simulink model "HPP"  (R2026a)
settings: Solver=ode1  StopTime=p.sim.Tstop  FixedStep=HPP_Tnet
model workspace (MAT data in the model file):
  HPP_Tnet = 0.001
  HPP_Ts = 0.001
  HPP_delays = 1
  HPP_f0 = 50
  HPP_network = 1
  HPP_simscape = 1
  buildInfo : object (value not decoded)
undefined symbols (not defined in the file): p
libraries: ee_lib x57, nesl_utility x29, fl_lib x6
(part 2 of 5)

== system HPP/HPP controller/P_set_bess to W link ==
  In1 : Inport
  gain 1 : Gain  Gain=p.ctrl.hppc.Pbase
  Out1 : Outport
  wires:
  In1/1 -> gain 1/1
  gain 1/1 -> Out1/1

== system HPP/HPP controller/P_set_spp to W link ==
  In1 : Inport
  gain 1 : Gain  Gain=p.ctrl.hppc.Pbase
  Out1 : Outport
  wires:
  In1/1 -> gain 1/1
  gain 1/1 -> Out1/1

== system HPP/HPP controller/P_set_wpp to W link ==
  In1 : Inport
  gain 1 : Gain  Gain=p.ctrl.hppc.Pbase
  Out1 : Outport
  wires:
  In1/1 -> gain 1/1
  gain 1/1 -> Out1/1

== system HPP/HPP controller/P_spp link ==
  In1 : Inport
  delay 3 : Subsystem  Description=Communication delay of p.comm.steps.meas_hppc steps, chosen per run: Fixed (HPP_delays = 1, length fixed at compile time, fastest) or Variable (HPP_delays = 2, tunable up to p.comm.maxDelay). See commParameters, comm.delays.  Variant=on
  gain 1 : Gain  Gain=1/p.ctrl.hppc.Pbase
  memory 2 : Memory
  Out1 : Outport
  wires:
  In1/1 -> gain 1/1
  memory 2/1 -> delay 3/1(u)
  gain 1/1 -> memory 2/1
  delay 3/1(y) -> Out1/1

== system HPP/HPP controller/P_wpp link ==
  In1 : Inport
  delay 3 : Subsystem  Description=Communication delay of p.comm.steps.meas_hppc steps, chosen per run: Fixed (HPP_delays = 1, length fixed at compile time, fastest) or Variable (HPP_delays = 2, tunable up to p.comm.maxDelay). See commParameters, comm.delays.  Variant=on
  gain 1 : Gain  Gain=1/p.ctrl.hppc.Pbase
  memory 2 : Memory
  Out1 : Outport
  wires:
  In1/1 -> gain 1/1
  delay 3/1(y) -> Out1/1
  memory 2/1 -> delay 3/1(u)
  gain 1/1 -> memory 2/1

== system HPP/HPP controller/Q_bess link ==
  In1 : Inport
  delay 3 : Subsystem  Description=Communication delay of p.comm.steps.meas_hppc steps, chosen per run: Fixed (HPP_delays = 1, length fixed at compile time, fastest) or Variable (HPP_delays = 2, tunable up to p.comm.maxDelay). See commParameters, comm.delays.  Variant=on
  gain 1 : Gain  Gain=1/p.ctrl.hppc.Pbase
  memory 2 : Memory
  Out1 : Outport
  wires:
  In1/1 -> gain 1/1
  gain 1/1 -> memory 2/1
  delay 3/1(y) -> Out1/1
  memory 2/1 -> delay 3/1(u)

== system HPP/HPP controller/Q_poc link ==
  In1 : Inport
  delay 3 : Subsystem  Description=Communication delay of p.comm.steps.meas_hppc steps, chosen per run: Fixed (HPP_delays = 1, length fixed at compile time, fastest) or Variable (HPP_delays = 2, tunable up to p.comm.maxDelay). See commParameters, comm.delays.  Variant=on
  gain 1 : Gain  Gain=1/p.ctrl.hppc.Pbase
  memory 2 : Memory
  Out1 : Outport
  wires:
  In1/1 -> gain 1/1
  delay 3/1(y) -> Out1/1
  memory 2/1 -> delay 3/1(u)
  gain 1/1 -> memory 2/1

== system HPP/HPP controller/Q_ref link ==
  In1 : Inport
  delay 2 : Subsystem  Description=Communication delay of p.comm.steps.tso steps, chosen per run: Fixed (HPP_delays = 1, length fixed at compile time, fastest) or Variable (HPP_delays = 2, tunable up to p.comm.maxDelay). See commParameters, comm.delays.  Variant=on
  gain 1 : Gain  Gain=1/p.ctrl.hppc.Pbase
  Out1 : Outport
  wires:
  In1/1 -> gain 1/1
  gain 1/1 -> delay 2/1(u)
  delay 2/1(y) -> Out1/1

== system HPP/HPP controller/Q_sat_bess link ==
  In1 : Inport
  delay 2 : Subsystem  Description=Communication delay of p.comm.steps.meas_hppc steps, chosen per run: Fixed (HPP_delays = 1, length fixed at compile time, fastest) or Variable (HPP_delays = 2, tunable up to p.comm.maxDelay). See commParameters, comm.delays.  Variant=on
  memory 1 : Memory
  Out1 : Outport
  wires:
  In1/1 -> memory 1/1
  delay 2/1(y) -> Out1/1
  memory 1/1 -> delay 2/1(u)

== system HPP/HPP controller/Q_sat_spp link ==
  In1 : Inport
  delay 2 : Subsystem  Description=Communication delay of p.comm.steps.meas_hppc steps, chosen per run: Fixed (HPP_delays = 1, length fixed at compile time, fastest) or Variable (HPP_delays = 2, tunable up to p.comm.maxDelay). See commParameters, comm.delays.  Variant=on
  memory 1 : Memory
  Out1 : Outport
  wires:
  In1/1 -> memory 1/1
  delay 2/1(y) -> Out1/1
  memory 1/1 -> delay 2/1(u)

== system HPP/HPP controller/Q_sat_wpp link ==
  In1 : Inport
  delay 2 : Subsystem  Description=Communication delay of p.comm.steps.meas_hppc steps, chosen per run: Fixed (HPP_delays = 1, length fixed at compile time, fastest) or Variable (HPP_delays = 2, tunable up to p.comm.maxDelay). See commParameters, comm.delays.  Variant=on
  memory 1 : Memory
  Out1 : Outport
  wires:
  In1/1 -> memory 1/1
  delay 2/1(y) -> Out1/1
  memory 1/1 -> delay 2/1(u)

== system HPP/HPP controller/Q_set_bess to var link ==
  In1 : Inport
  gain 1 : Gain  Gain=p.ctrl.hppc.Pbase
  Out1 : Outport
  wires:
  In1/1 -> gain 1/1
  gain 1/1 -> Out1/1

== system HPP/HPP controller/Q_set_spp to var link ==
  In1 : Inport
  gain 1 : Gain  Gain=p.ctrl.hppc.Pbase
  Out1 : Outport
  wires:
  In1/1 -> gain 1/1
  gain 1/1 -> Out1/1

== system HPP/HPP controller/Q_set_wpp to var link ==
  In1 : Inport
  gain 1 : Gain  Gain=p.ctrl.hppc.Pbase
  Out1 : Outport
  wires:
  In1/1 -> gain 1/1
  gain 1/1 -> Out1/1

== system HPP/HPP controller/Q_spp link ==
  In1 : Inport
  delay 3 : Subsystem  Description=Communication delay of p.comm.steps.meas_hppc steps, chosen per run: Fixed (HPP_delays = 1, length fixed at compile time, fastest) or Variable (HPP_delays = 2, tunable up to p.comm.maxDelay). See commParameters, comm.delays.  Variant=on
  gain 1 : Gain  Gain=1/p.ctrl.hppc.Pbase
  memory 2 : Memory
  Out1 : Outport
  wires:
  In1/1 -> gain 1/1
  delay 3/1(y) -> Out1/1
  memory 2/1 -> delay 3/1(u)
  gain 1/1 -> memory 2/1

== system HPP/HPP controller/Q_wpp link ==
  In1 : Inport
  delay 3 : Subsystem  Description=Communication delay of p.comm.steps.meas_hppc steps, chosen per run: Fixed (HPP_delays = 1, length fixed at compile time, fastest) or Variable (HPP_delays = 2, tunable up to p.comm.maxDelay). See commParameters, comm.delays.  Variant=on
  gain 1 : Gain  Gain=1/p.ctrl.hppc.Pbase
  memory 2 : Memory
  Out1 : Outport
  wires:
  In1/1 -> gain 1/1
  memory 2/1 -> delay 3/1(u)
  gain 1/1 -> memory 2/1
  delay 3/1(y) -> Out1/1

== system HPP/HPP controller/SOC_bess link ==
  In1 : Inport
  delay 2 : Subsystem  Description=Communication delay of p.comm.steps.meas_hppc steps, chosen per run: Fixed (HPP_delays = 1, length fixed at compile time, fastest) or Variable (HPP_delays = 2, tunable up to p.comm.maxDelay). See commParameters, comm.delays.  Variant=on
  memory 1 : Memory
  Out1 : Outport
  wires:
  In1/1 -> memory 1/1
  delay 2/1(y) -> Out1/1
  memory 1/1 -> delay 2/1(u)

== system HPP/HPP controller/V_poc link ==
  In1 : Inport
  delay 2 : Subsystem  Description=Communication delay of p.comm.steps.meas_hppc steps, chosen per run: Fixed (HPP_delays = 1, length fixed at compile time, fastest) or Variable (HPP_delays = 2, tunable up to p.comm.maxDelay). See commParameters, comm.delays.  Variant=on
  memory 1 : Memory
  Out1 : Outport
  wires:
  In1/1 -> memory 1/1
  memory 1/1 -> delay 2/1(u)
  delay 2/1(y) -> Out1/1

== system HPP/Network/Grid frequency ==
  POC meas : Inport
  1 + w : Bias  Bias=1  SaturateOnIntegerOverflow=off
  HPP change : Subsystem  Description=dPh = (P_poc - P_hold) / Ssys; P_hold follows P_poc until tOn (system balanced at tOn)
  POC sel : BusSelector  OutputSignals=P_poc
  P_poc[k-1] : UnitDelay  SampleTime=-1
  active : Subsystem  Description=swing equation on (swing = 1) and t >= tOn
  disturbance : Subsystem  Description=dP_dist = dist.dP for t >= dist.t0
  grid source angle : Subsystem  Description=th = wrap(th[k-1] + 2 pi f0 (f - 1) Ts); theta = wrap(th + dphi (t >= pjump.t0))
  imposed : Subsystem  Description=1 + fev.df (t >= fev.t0) + profile(t)
  swing : Constant  Value=g.sys.swing
  swing equation : Subsystem  Description=2H dw/dt = Pm + dPh - dP_dist - D w; governor and turbine (Pm); forward Euler from tOn
  swing? : Switch  Criteria=u2 > Threshold  Threshold=0.5  SaturateOnIntegerOverflow=off  InputSameDT=off
  t : DigitalClock  SampleTime=p.sim.Ts
  f : Outport
  theta : Outport  Port=2
  wires:
  POC meas/1 -> POC sel/1
  POC sel/1 -> P_poc[k-1]/1  "<P_poc>"
  P_poc[k-1]/1 -> HPP change/1(P_poc)  "P_poc"
  t/1 -> active/1(t), disturbance/1(t), imposed/1(t), grid source angle/2(t)  "t"
  active/1(active) -> HPP change/2(active), swing equation/3(active)  "active"
  HPP change/1(dPh) -> swing equation/1(dPh)  "dPh"
  disturbance/1(dPd) -> swing equation/2(dPd)  "dPd"
  swing equation/1(w) -> 1 + w/1  "w"
  1 + w/1 -> swing?/1
  swing/1 -> swing?/2
  imposed/1(f_imp) -> swing?/3  "f_imp"
  swing?/1 -> f/1, grid source angle/1(f)  "f"
  grid source angle/1(theta) -> theta/1  "theta"

== system HPP/Network/Network model ==
  note: 1) Add Subsystem or Model blocks as valid variant choices.
      | 2) You cannot connect blocks at this level. At simulation, connectivity is automatically
      | determined, based on the active variant and port name matching.
  I wpp : Inport
  I spp : Inport  Port=2
  I bess : Inport  Port=3
  f grid : Inport  Port=4
  theta : Inport  Port=5
  Nodal : Subsystem  VariantControl=HPP_network == 1  mask{net=p.net.solver}
      mask prompts: net "Network solver data"
      mask help: Positive-sequence phasor network (collector system, transformers, grid). Solves V = Z*I each step. Data from networkSolverData(p).
  Simscape : Subsystem  Description=Network as a Simscape Electrical model in phasor (frequency-and-time) or EMT mode (buildNetworkSimscape). Same ports as the nodal network. Electrical nodes are joined by Connection Labels (collector, tap, HPP bus, POC); signals by local Goto/From.  VariantControl=HPP_network == 2
  network : Outport
  POC meas : Outport  Port=2

== system HPP/PV plant/I_im to system pu link ==
  In1 : Inport
  gain 1 : Gain  Gain=p.ctrl.pv.Pbase/p.grid.Pbase
  Out1 : Outport
  wires:
  gain 1/1 -> Out1/1
  In1/1 -> gain 1/1

== system HPP/PV plant/I_re to system pu link ==
  In1 : Inport
  gain 1 : Gain  Gain=p.ctrl.pv.Pbase/p.grid.Pbase
  Out1 : Outport
  wires:
  In1/1 -> gain 1/1
  gain 1/1 -> Out1/1

== system HPP/PV plant/P to W link ==
  In1 : Inport
  gain 1 : Gain  Gain=p.ctrl.sppc.Pbase
  Out1 : Outport
  wires:
  gain 1/1 -> Out1/1
  In1/1 -> gain 1/1

== system HPP/PV plant/P_avail to W link ==
  In1 : Inport
  gain 1 : Gain  Gain=p.ctrl.sppc.Pbase
  Out1 : Outport
  wires:
  gain 1/1 -> Out1/1
  In1/1 -> gain 1/1

== system HPP/PV plant/P_avail_k link ==
  In1 : Inport
  delay 3 : Subsystem  Description=Communication delay of p.comm.steps.meas_plant steps, chosen per run: Fixed (HPP_delays = 1, length fixed at compile time, fastest) or Variable (HPP_delays = 2, tunable up to p.comm.maxDelay). See commParameters, comm.delays.  Variant=on
  gain 1 : Gain  Gain=p.ctrl.pv.Pbase/p.ctrl.sppc.Pbase
  memory 2 : Memory
  Out1 : Outport
  wires:
  In1/1 -> gain 1/1
  gain 1/1 -> memory 2/1
  memory 2/1 -> delay 3/1(u)
  delay 3/1(y) -> Out1/1

== system HPP/PV plant/P_meas link ==
  In1 : Inport
  delay 3 : Subsystem  Description=Communication delay of p.comm.steps.meas_plant steps, chosen per run: Fixed (HPP_delays = 1, length fixed at compile time, fastest) or Variable (HPP_delays = 2, tunable up to p.comm.maxDelay). See commParameters, comm.delays.  Variant=on
  gain 1 : Gain  Gain=1/p.ctrl.sppc.Pbase
  memory 2 : Memory
  Out1 : Outport
  wires:
  In1/1 -> gain 1/1
  gain 1/1 -> memory 2/1
  memory 2/1 -> delay 3/1(u)
  delay 3/1(y) -> Out1/1

== system HPP/PV plant/P_set link ==
  In1 : Inport
  delay 1 : Subsystem  Description=Communication delay of p.comm.steps.hppc_to_plant steps, chosen per run: Fixed (HPP_delays = 1, length fixed at compile time, fastest) or Variable (HPP_delays = 2, tunable up to p.comm.maxDelay). See commParameters, comm.delays.  Variant=on
  gain 2 : Gain  Gain=1/p.ctrl.sppc.Pbase
  Out1 : Outport
  wires:
  In1/1 -> delay 1/1(u)
  delay 1/1(y) -> gain 2/1
  gain 2/1 -> Out1/1

== system HPP/PV plant/P_set_k link ==
  In1 : Inport
  delay 1 : Subsystem  Description=Communication delay of p.comm.steps.plant_to_asset steps, chosen per run: Fixed (HPP_delays = 1, length fixed at compile time, fastest) or Variable (HPP_delays = 2, tunable up to p.comm.maxDelay). See commParameters, comm.delays.  Variant=on
  gain 2 : Gain  Gain=p.ctrl.sppc.Pbase/p.ctrl.pv.Pbase
  Out1 : Outport
  wires:
  In1/1 -> delay 1/1(u)
  delay 1/1(y) -> gain 2/1
  gain 2/1 -> Out1/1

== system HPP/PV plant/Q to W link ==
  In1 : Inport
  gain 1 : Gain  Gain=p.ctrl.sppc.Pbase
  Out1 : Outport
  wires:
  gain 1/1 -> Out1/1
  In1/1 -> gain 1/1

== system HPP/PV plant/Q_meas link ==
  In1 : Inport
  delay 3 : Subsystem  Description=Communication delay of p.comm.steps.meas_plant steps, chosen per run: Fixed (HPP_delays = 1, length fixed at compile time, fastest) or Variable (HPP_delays = 2, tunable up to p.comm.maxDelay). See commParameters, comm.delays.  Variant=on
  gain 1 : Gain  Gain=1/p.ctrl.sppc.Pbase
  memory 2 : Memory
  Out1 : Outport
  wires:
  In1/1 -> gain 1/1
  gain 1/1 -> memory 2/1
  memory 2/1 -> delay 3/1(u)
  delay 3/1(y) -> Out1/1

== system HPP/PV plant/Q_set link ==
  In1 : Inport
  delay 1 : Subsystem  Description=Communication delay of p.comm.steps.hppc_to_plant steps, chosen per run: Fixed (HPP_delays = 1, length fixed at compile time, fastest) or Variable (HPP_delays = 2, tunable up to p.comm.maxDelay). See commParameters, comm.delays.  Variant=on
  gain 2 : Gain  Gain=1/p.ctrl.sppc.Pbase
  Out1 : Outport
  wires:
  delay 1/1(y) -> gain 2/1
  In1/1 -> delay 1/1(u)
  gain 2/1 -> Out1/1

== system HPP/PV plant/Q_set_k link ==
  In1 : Inport
  delay 1 : Subsystem  Description=Communication delay of p.comm.steps.plant_to_asset steps, chosen per run: Fixed (HPP_delays = 1, length fixed at compile time, fastest) or Variable (HPP_delays = 2, tunable up to p.comm.maxDelay). See commParameters, comm.delays.  Variant=on
  gain 2 : Gain  Gain=p.ctrl.sppc.Pbase/p.ctrl.pv.Pbase
  Out1 : Outport
  wires:
  In1/1 -> delay 1/1(u)
  delay 1/1(y) -> gain 2/1
  gain 2/1 -> Out1/1

== system HPP/PV plant/V_meas link ==
  In1 : Inport
  delay 2 : Subsystem  Description=Communication delay of p.comm.steps.meas_plant steps, chosen per run: Fixed (HPP_delays = 1, length fixed at compile time, fastest) or Variable (HPP_delays = 2, tunable up to p.comm.maxDelay). See commParameters, comm.delays.  Variant=on
  memory 1 : Memory
  Out1 : Outport
  wires:
  In1/1 -> memory 1/1
  delay 2/1(y) -> Out1/1
  memory 1/1 -> delay 2/1(u)

== system HPP/PV plant/f_meas link ==
  In1 : Inport
  memory 1 : Memory
  Out1 : Outport
  wires:
  memory 1/1 -> Out1/1
  In1/1 -> memory 1/1

== system HPP/Wind plant/I_im to system pu link ==
  In1 : Inport
  gain 1 : Gain  Gain=p.ctrl.wt.Pbase/p.grid.Pbase
  Out1 : Outport
  wires:
  In1/1 -> gain 1/1
  gain 1/1 -> Out1/1

== system HPP/Wind plant/I_re to system pu link ==
  In1 : Inport
  gain 1 : Gain  Gain=p.ctrl.wt.Pbase/p.grid.Pbase
  Out1 : Outport
  wires:
  In1/1 -> gain 1/1
  gain 1/1 -> Out1/1

== system HPP/Wind plant/P to W link ==
  In1 : Inport
  gain 1 : Gain  Gain=p.ctrl.wppc.Pbase
  Out1 : Outport
  wires:
  gain 1/1 -> Out1/1
  In1/1 -> gain 1/1

== system HPP/Wind plant/P_avail to W link ==
  In1 : Inport
  gain 1 : Gain  Gain=p.ctrl.wppc.Pbase
  Out1 : Outport
  wires:
  gain 1/1 -> Out1/1
  In1/1 -> gain 1/1

== system HPP/Wind plant/P_avail_k link ==
  In1 : Inport
  delay 3 : Subsystem  Description=Communication delay of p.comm.steps.meas_plant steps, chosen per run: Fixed (HPP_delays = 1, length fixed at compile time, fastest) or Variable (HPP_delays = 2, tunable up to p.comm.maxDelay). See commParameters, comm.delays.  Variant=on
  gain 1 : Gain  Gain=p.ctrl.wt.Pbase/p.ctrl.wppc.Pbase
  memory 2 : Memory
  Out1 : Outport
  wires:
  In1/1 -> gain 1/1
  gain 1/1 -> memory 2/1
  memory 2/1 -> delay 3/1(u)
  delay 3/1(y) -> Out1/1

== system HPP/Wind plant/P_meas link ==
  In1 : Inport
  delay 3 : Subsystem  Description=Communication delay of p.comm.steps.meas_plant steps, chosen per run: Fixed (HPP_delays = 1, length fixed at compile time, fastest) or Variable (HPP_delays = 2, tunable up to p.comm.maxDelay). See commParameters, comm.delays.  Variant=on
  gain 1 : Gain  Gain=1/p.ctrl.wppc.Pbase
  memory 2 : Memory
  Out1 : Outport
  wires:
  In1/1 -> gain 1/1
  gain 1/1 -> memory 2/1
  memory 2/1 -> delay 3/1(u)
  delay 3/1(y) -> Out1/1

== system HPP/Wind plant/P_set link ==
  In1 : Inport
  delay 1 : Subsystem  Description=Communication delay of p.comm.steps.hppc_to_plant steps, chosen per run: Fixed (HPP_delays = 1, length fixed at compile time, fastest) or Variable (HPP_delays = 2, tunable up to p.comm.maxDelay). See commParameters, comm.delays.  Variant=on
  gain 2 : Gain  Gain=1/p.ctrl.wppc.Pbase
  Out1 : Outport
  wires:
  In1/1 -> delay 1/1(u)
  delay 1/1(y) -> gain 2/1
  gain 2/1 -> Out1/1

== system HPP/Wind plant/P_set_k link ==
  In1 : Inport
  delay 1 : Subsystem  Description=Communication delay of p.comm.steps.plant_to_asset steps, chosen per run: Fixed (HPP_delays = 1, length fixed at compile time, fastest) or Variable (HPP_delays = 2, tunable up to p.comm.maxDelay). See commParameters, comm.delays.  Variant=on
  gain 2 : Gain  Gain=p.ctrl.wppc.Pbase/p.ctrl.wt.Pbase
  Out1 : Outport
  wires:
  In1/1 -> delay 1/1(u)
  delay 1/1(y) -> gain 2/1
  gain 2/1 -> Out1/1

== system HPP/Wind plant/Q to W link ==
  In1 : Inport
  gain 1 : Gain  Gain=p.ctrl.wppc.Pbase
  Out1 : Outport
  wires:
  In1/1 -> gain 1/1
  gain 1/1 -> Out1/1

== system HPP/Wind plant/Q_meas link ==
  In1 : Inport
  delay 3 : Subsystem  Description=Communication delay of p.comm.steps.meas_plant steps, chosen per run: Fixed (HPP_delays = 1, length fixed at compile time, fastest) or Variable (HPP_delays = 2, tunable up to p.comm.maxDelay). See commParameters, comm.delays.  Variant=on
  gain 1 : Gain  Gain=1/p.ctrl.wppc.Pbase
  memory 2 : Memory
  Out1 : Outport
  wires:
  In1/1 -> gain 1/1
  gain 1/1 -> memory 2/1
  memory 2/1 -> delay 3/1(u)
  delay 3/1(y) -> Out1/1

== system HPP/Wind plant/Q_set link ==
  In1 : Inport
  delay 1 : Subsystem  Description=Communication delay of p.comm.steps.hppc_to_plant steps, chosen per run: Fixed (HPP_delays = 1, length fixed at compile time, fastest) or Variable (HPP_delays = 2, tunable up to p.comm.maxDelay). See commParameters, comm.delays.  Variant=on
  gain 2 : Gain  Gain=1/p.ctrl.wppc.Pbase
  Out1 : Outport
  wires:
  In1/1 -> delay 1/1(u)
  delay 1/1(y) -> gain 2/1
  gain 2/1 -> Out1/1

== system HPP/Wind plant/Q_set_k link ==
  In1 : Inport
  delay 1 : Subsystem  Description=Communication delay of p.comm.steps.plant_to_asset steps, chosen per run: Fixed (HPP_delays = 1, length fixed at compile time, fastest) or Variable (HPP_delays = 2, tunable up to p.comm.maxDelay). See commParameters, comm.delays.  Variant=on
  gain 2 : Gain  Gain=p.ctrl.wppc.Pbase/p.ctrl.wt.Pbase
  Out1 : Outport
  wires:
  In1/1 -> delay 1/1(u)
  delay 1/1(y) -> gain 2/1
  gain 2/1 -> Out1/1

== system HPP/Wind plant/V_meas link ==
  In1 : Inport
  delay 2 : Subsystem  Description=Communication delay of p.comm.steps.meas_plant steps, chosen per run: Fixed (HPP_delays = 1, length fixed at compile time, fastest) or Variable (HPP_delays = 2, tunable up to p.comm.maxDelay). See commParameters, comm.delays.  Variant=on
  memory 1 : Memory
  Out1 : Outport
  wires:
  In1/1 -> memory 1/1
  memory 1/1 -> delay 2/1(u)
  delay 2/1(y) -> Out1/1

== system HPP/Wind plant/f_meas link ==
  In1 : Inport
  memory 1 : Memory
  Out1 : Outport
  wires:
  In1/1 -> memory 1/1
  memory 1/1 -> Out1/1

== system HPP/BESS plant/P_avail_k link/delay 3 ==
  note: 1) Add Subsystem or Model blocks as valid variant choices.
      | 2) You cannot connect blocks at this level. At simulation, connectivity is automatically
      | determined, based on the active variant and port name matching.
  u : Inport
  Fixed : Subsystem  VariantControl=HPP_delays == 1
  Variable : Subsystem  VariantControl=HPP_delays == 2
  y : Outport

== system HPP/BESS plant/P_meas link/delay 3 ==
  note: 1) Add Subsystem or Model blocks as valid variant choices.
      | 2) You cannot connect blocks at this level. At simulation, connectivity is automatically
      | determined, based on the active variant and port name matching.
  u : Inport
  Fixed : Subsystem  VariantControl=HPP_delays == 1
  Variable : Subsystem  VariantControl=HPP_delays == 2
  y : Outport

== system HPP/BESS plant/P_set link/delay 1 ==
  note: 1) Add Subsystem or Model blocks as valid variant choices.
      | 2) You cannot connect blocks at this level. At simulation, connectivity is automatically
      | determined, based on the active variant and port name matching.
  u : Inport
  Fixed : Subsystem  VariantControl=HPP_delays == 1
  Variable : Subsystem  VariantControl=HPP_delays == 2
  y : Outport

== system HPP/BESS plant/P_set_k link/delay 1 ==
  note: 1) Add Subsystem or Model blocks as valid variant choices.
      | 2) You cannot connect blocks at this level. At simulation, connectivity is automatically
      | determined, based on the active variant and port name matching.
  u : Inport
  Fixed : Subsystem  VariantControl=HPP_delays == 1
  Variable : Subsystem  VariantControl=HPP_delays == 2
  y : Outport

== system HPP/BESS plant/Q_meas link/delay 3 ==
  note: 1) Add Subsystem or Model blocks as valid variant choices.
      | 2) You cannot connect blocks at this level. At simulation, connectivity is automatically
      | determined, based on the active variant and port name matching.
  u : Inport
  Fixed : Subsystem  VariantControl=HPP_delays == 1
  Variable : Subsystem  VariantControl=HPP_delays == 2
  y : Outport

== system HPP/BESS plant/Q_set link/delay 1 ==
  note: 1) Add Subsystem or Model blocks as valid variant choices.
      | 2) You cannot connect blocks at this level. At simulation, connectivity is automatically
      | determined, based on the active variant and port name matching.
  u : Inport
  Fixed : Subsystem  VariantControl=HPP_delays == 1
  Variable : Subsystem  VariantControl=HPP_delays == 2
  y : Outport

== system HPP/BESS plant/Q_set_k link/delay 1 ==
  note: 1) Add Subsystem or Model blocks as valid variant choices.
      | 2) You cannot connect blocks at this level. At simulation, connectivity is automatically
      | determined, based on the active variant and port name matching.
  u : Inport
  Fixed : Subsystem  VariantControl=HPP_delays == 1
  Variable : Subsystem  VariantControl=HPP_delays == 2
  y : Outport

== system HPP/BESS plant/SOC_k link/delay 2 ==
  note: 1) Add Subsystem or Model blocks as valid variant choices.
      | 2) You cannot connect blocks at this level. At simulation, connectivity is automatically
      | determined, based on the active variant and port name matching.
  u : Inport
  Fixed : Subsystem  VariantControl=HPP_delays == 1
  Variable : Subsystem  VariantControl=HPP_delays == 2
  y : Outport

== system HPP/BESS plant/V_meas link/delay 2 ==
  note: 1) Add Subsystem or Model blocks as valid variant choices.
      | 2) You cannot connect blocks at this level. At simulation, connectivity is automatically
      | determined, based on the active variant and port name matching.
  u : Inport
  Fixed : Subsystem  VariantControl=HPP_delays == 1
  Variable : Subsystem  VariantControl=HPP_delays == 2
  y : Outport

== system HPP/HPP controller/P_avail_spp link/delay 3 ==
  note: 1) Add Subsystem or Model blocks as valid variant choices.
      | 2) You cannot connect blocks at this level. At simulation, connectivity is automatically
      | determined, based on the active variant and port name matching.
  u : Inport
  Fixed : Subsystem  VariantControl=HPP_delays == 1
  Variable : Subsystem  VariantControl=HPP_delays == 2
  y : Outport

== system HPP/HPP controller/P_avail_wpp link/delay 3 ==
  note: 1) Add Subsystem or Model blocks as valid variant choices.
      | 2) You cannot connect blocks at this level. At simulation, connectivity is automatically
      | determined, based on the active variant and port name matching.
  u : Inport
  Fixed : Subsystem  VariantControl=HPP_delays == 1
  Variable : Subsystem  VariantControl=HPP_delays == 2
  y : Outport

== system HPP/HPP controller/P_bess link/delay 3 ==
  note: 1) Add Subsystem or Model blocks as valid variant choices.
      | 2) You cannot connect blocks at this level. At simulation, connectivity is automatically
      | determined, based on the active variant and port name matching.
  u : Inport
  Fixed : Subsystem  VariantControl=HPP_delays == 1
  Variable : Subsystem  VariantControl=HPP_delays == 2
  y : Outport

== system HPP/HPP controller/P_chg_max_bess link/delay 3 ==
  note: 1) Add Subsystem or Model blocks as valid variant choices.
      | 2) You cannot connect blocks at this level. At simulation, connectivity is automatically
      | determined, based on the active variant and port name matching.
  u : Inport
  Fixed : Subsystem  VariantControl=HPP_delays == 1
  Variable : Subsystem  VariantControl=HPP_delays == 2
  y : Outport

== system HPP/HPP controller/P_dis_max_bess link/delay 3 ==
  note: 1) Add Subsystem or Model blocks as valid variant choices.
      | 2) You cannot connect blocks at this level. At simulation, connectivity is automatically
      | determined, based on the active variant and port name matching.
  u : Inport
  Fixed : Subsystem  VariantControl=HPP_delays == 1
  Variable : Subsystem  VariantControl=HPP_delays == 2
  y : Outport

== system HPP/HPP controller/P_poc link/delay 3 ==
  note: 1) Add Subsystem or Model blocks as valid variant choices.
      | 2) You cannot connect blocks at this level. At simulation, connectivity is automatically
      | determined, based on the active variant and port name matching.
  u : Inport
  Fixed : Subsystem  VariantControl=HPP_delays == 1
  Variable : Subsystem  VariantControl=HPP_delays == 2
  y : Outport

== system HPP/HPP controller/P_ref link/delay 2 ==
  note: 1) Add Subsystem or Model blocks as valid variant choices.
      | 2) You cannot connect blocks at this level. At simulation, connectivity is automatically
      | determined, based on the active variant and port name matching.
  u : Inport
  Fixed : Subsystem  VariantControl=HPP_delays == 1
  Variable : Subsystem  VariantControl=HPP_delays == 2
  y : Outport

== system HPP/HPP controller/P_spp link/delay 3 ==
  note: 1) Add Subsystem or Model blocks as valid variant choices.
      | 2) You cannot connect blocks at this level. At simulation, connectivity is automatically
      | determined, based on the active variant and port name matching.
  u : Inport
  Fixed : Subsystem  VariantControl=HPP_delays == 1
  Variable : Subsystem  VariantControl=HPP_delays == 2
  y : Outport

== system HPP/HPP controller/P_wpp link/delay 3 ==
  note: 1) Add Subsystem or Model blocks as valid variant choices.
      | 2) You cannot connect blocks at this level. At simulation, connectivity is automatically
      | determined, based on the active variant and port name matching.
  u : Inport
  Fixed : Subsystem  VariantControl=HPP_delays == 1
  Variable : Subsystem  VariantControl=HPP_delays == 2
  y : Outport

== system HPP/HPP controller/Q_bess link/delay 3 ==
  note: 1) Add Subsystem or Model blocks as valid variant choices.
      | 2) You cannot connect blocks at this level. At simulation, connectivity is automatically
      | determined, based on the active variant and port name matching.
  u : Inport
  Fixed : Subsystem  VariantControl=HPP_delays == 1
  Variable : Subsystem  VariantControl=HPP_delays == 2
  y : Outport

== system HPP/HPP controller/Q_poc link/delay 3 ==
  note: 1) Add Subsystem or Model blocks as valid variant choices.
      | 2) You cannot connect blocks at this level. At simulation, connectivity is automatically
      | determined, based on the active variant and port name matching.
  u : Inport
  Fixed : Subsystem  VariantControl=HPP_delays == 1
  Variable : Subsystem  VariantControl=HPP_delays == 2
  y : Outport

== system HPP/HPP controller/Q_ref link/delay 2 ==
  note: 1) Add Subsystem or Model blocks as valid variant choices.
      | 2) You cannot connect blocks at this level. At simulation, connectivity is automatically
      | determined, based on the active variant and port name matching.
  u : Inport
  Fixed : Subsystem  VariantControl=HPP_delays == 1
  Variable : Subsystem  VariantControl=HPP_delays == 2
  y : Outport

== system HPP/HPP controller/Q_sat_bess link/delay 2 ==
  note: 1) Add Subsystem or Model blocks as valid variant choices.
      | 2) You cannot connect blocks at this level. At simulation, connectivity is automatically
      | determined, based on the active variant and port name matching.
  u : Inport
  Fixed : Subsystem  VariantControl=HPP_delays == 1
  Variable : Subsystem  VariantControl=HPP_delays == 2
  y : Outport

== system HPP/HPP controller/Q_sat_spp link/delay 2 ==
  note: 1) Add Subsystem or Model blocks as valid variant choices.
      | 2) You cannot connect blocks at this level. At simulation, connectivity is automatically
      | determined, based on the active variant and port name matching.
  u : Inport
  Fixed : Subsystem  VariantControl=HPP_delays == 1
  Variable : Subsystem  VariantControl=HPP_delays == 2
  y : Outport

== system HPP/HPP controller/Q_sat_wpp link/delay 2 ==
  note: 1) Add Subsystem or Model blocks as valid variant choices.
      | 2) You cannot connect blocks at this level. At simulation, connectivity is automatically
      | determined, based on the active variant and port name matching.
  u : Inport
  Fixed : Subsystem  VariantControl=HPP_delays == 1
  Variable : Subsystem  VariantControl=HPP_delays == 2
  y : Outport

== system HPP/HPP controller/Q_spp link/delay 3 ==
  note: 1) Add Subsystem or Model blocks as valid variant choices.
      | 2) You cannot connect blocks at this level. At simulation, connectivity is automatically
      | determined, based on the active variant and port name matching.
  u : Inport
  Fixed : Subsystem  VariantControl=HPP_delays == 1
  Variable : Subsystem  VariantControl=HPP_delays == 2
  y : Outport

== system HPP/HPP controller/Q_wpp link/delay 3 ==
  note: 1) Add Subsystem or Model blocks as valid variant choices.
      | 2) You cannot connect blocks at this level. At simulation, connectivity is automatically
      | determined, based on the active variant and port name matching.
  u : Inport
  Fixed : Subsystem  VariantControl=HPP_delays == 1
  Variable : Subsystem  VariantControl=HPP_delays == 2
  y : Outport

== system HPP/HPP controller/SOC_bess link/delay 2 ==
  note: 1) Add Subsystem or Model blocks as valid variant choices.
      | 2) You cannot connect blocks at this level. At simulation, connectivity is automatically
      | determined, based on the active variant and port name matching.
  u : Inport
  Fixed : Subsystem  VariantControl=HPP_delays == 1
  Variable : Subsystem  VariantControl=HPP_delays == 2
  y : Outport

== system HPP/HPP controller/V_poc link/delay 2 ==
  note: 1) Add Subsystem or Model blocks as valid variant choices.
      | 2) You cannot connect blocks at this level. At simulation, connectivity is automatically
      | determined, based on the active variant and port name matching.
  u : Inport
  Fixed : Subsystem  VariantControl=HPP_delays == 1
  Variable : Subsystem  VariantControl=HPP_delays == 2
  y : Outport

== system HPP/Network/Grid frequency/HPP change ==
  P_poc : Inport
  active : Inport  Port=2
  P_hold[k-1] : Delay  DelayLength=1  InitialConditionSource=Input port
      settings: InputPortMap=u0,p4
  P_poc - P_hold : Sum  Inputs=+-
  Ssys : Constant  Value=g.sys.Ssys
  hold? : Switch  Criteria=u2 ~= 0  SaturateOnIntegerOverflow=off  InputSameDT=off
  ÷ Ssys : Product  Inputs=*/
  dPh : Outport
  wires:
  P_hold[k-1]/1 -> hold?/1
  active/1 -> hold?/2
  P_poc/1 -> hold?/3, P_hold[k-1]/2, P_poc - P_hold/1
  hold?/1 -> P_hold[k-1]/1, P_poc - P_hold/2  "P_hold"
  P_poc - P_hold/1 -> ÷ Ssys/1
  Ssys/1 -> ÷ Ssys/2
  ÷ Ssys/1 -> dPh/1

== system HPP/Network/Grid frequency/active ==
  t : Inport
  0.5 : Constant  Value=0.5
  and : Logic  AllPortsSameDT=off  OutDataTypeStr=boolean
  swing : Constant  Value=g.sys.swing
  swing > 0.5 : RelationalOperator  Operator=>  OutDataTypeStr=boolean  RndMeth=Simplest  InputSameDT=off
  t >= tOn : RelationalOperator  OutDataTypeStr=boolean  RndMeth=Simplest  InputSameDT=off
  tOn : Constant  Value=g.sys.tOn
  active : Outport
  wires:
  t/1 -> t >= tOn/1
  tOn/1 -> t >= tOn/2
  swing/1 -> swing > 0.5/1
  0.5/1 -> swing > 0.5/2
  t >= tOn/1 -> and/1
  swing > 0.5/1 -> and/2
  and/1 -> active/1

== system HPP/Network/Grid frequency/disturbance ==
  t : Inport
  dP : Gain  Gain=g.sys.dist.dP
  dist t0 : Constant  Value=g.sys.dist.t0
  on : DataTypeConversion  OutDataTypeStr=double  SaturateOnIntegerOverflow=off  RndMeth=Floor
  t >= t0 : RelationalOperator  OutDataTypeStr=boolean  RndMeth=Simplest  InputSameDT=off
  dPd : Outport
  wires:
  t/1 -> t >= t0/1
  dist t0/1 -> t >= t0/2
  t >= t0/1 -> on/1
  on/1 -> dP/1
  dP/1 -> dPd/1

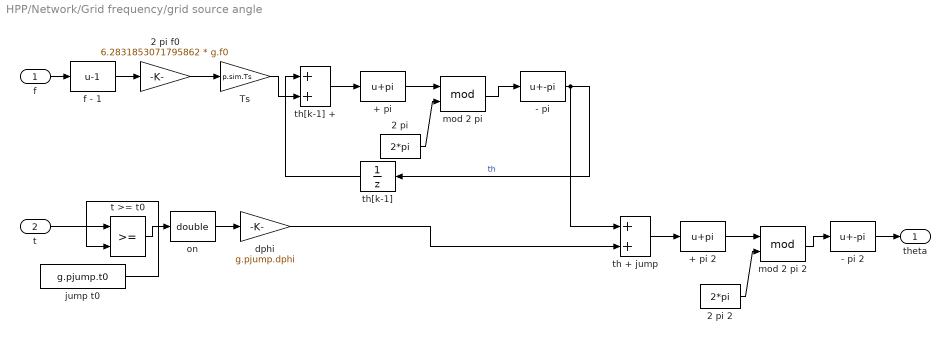
== system HPP/Network/Grid frequency/grid source angle ==
  f : Inport
  t : Inport  Port=2
  + pi : Bias  Bias=pi  SaturateOnIntegerOverflow=off
  + pi 2 : Bias  Bias=pi  SaturateOnIntegerOverflow=off
  - pi : Bias  Bias=-pi  SaturateOnIntegerOverflow=off
  - pi 2 : Bias  Bias=-pi  SaturateOnIntegerOverflow=off
  2 pi : Constant  Value=2*pi
  2 pi 2 : Constant  Value=2*pi
  2 pi f0 : Gain  Gain=6.2831853071795862 * g.f0
  Ts : Gain  Gain=p.sim.Ts
  dphi : Gain  Gain=g.pjump.dphi
  f - 1 : Bias  Bias=-1  SaturateOnIntegerOverflow=off
  jump t0 : Constant  Value=g.pjump.t0
  mod 2 pi : Math  Operator=mod
  mod 2 pi 2 : Math  Operator=mod
  on : DataTypeConversion  OutDataTypeStr=double  SaturateOnIntegerOverflow=off  RndMeth=Floor
  t >= t0 : RelationalOperator  OutDataTypeStr=boolean  RndMeth=Simplest  InputSameDT=off
  th + jump : Sum
  th[k-1] : UnitDelay  SampleTime=-1
  th[k-1] + : Sum
  theta : Outport
  wires:
  f/1 -> f - 1/1
  f - 1/1 -> 2 pi f0/1
  2 pi f0/1 -> Ts/1
  th[k-1]/1 -> th[k-1] +/1
  Ts/1 -> th[k-1] +/2
  th[k-1] +/1 -> + pi/1
  + pi/1 -> mod 2 pi/1
  2 pi/1 -> mod 2 pi/2
  mod 2 pi/1 -> - pi/1
  - pi/1 -> th[k-1]/1, th + jump/1  "th"
  t/1 -> t >= t0/1
  jump t0/1 -> t >= t0/2
  t >= t0/1 -> on/1
  on/1 -> dphi/1
  dphi/1 -> th + jump/2
  th + jump/1 -> + pi 2/1
  + pi 2/1 -> mod 2 pi 2/1
  2 pi 2/1 -> mod 2 pi 2/2
  mod 2 pi 2/1 -> - pi 2/1
  - pi 2/1 -> theta/1

== system HPP/Network/Grid frequency/imposed ==
  t : Inport
  + profile : Sum
  1 + : Bias  Bias=1  SaturateOnIntegerOverflow=off
  df : Gain  Gain=g.fev.df
  fev t0 : Constant  Value=g.fev.t0
  on : DataTypeConversion  OutDataTypeStr=double  SaturateOnIntegerOverflow=off  RndMeth=Floor
  profile : Lookup_n-D  NumberOfTableDimensions=1  BreakpointsForDimension1=g.fprof.t  Table=g.fprof.df  ExtrapMethod=Clip  InternalRulePriority=Speed  RndMeth=Simplest
  t >= t0 : RelationalOperator  OutDataTypeStr=boolean  RndMeth=Simplest  InputSameDT=off
  f_imp : Outport
  wires:
  t/1 -> t >= t0/1, profile/1
  fev t0/1 -> t >= t0/2
  t >= t0/1 -> on/1
  on/1 -> df/1
  df/1 -> 1 +/1
  1 +/1 -> + profile/1
  profile/1 -> + profile/2
  + profile/1 -> f_imp/1

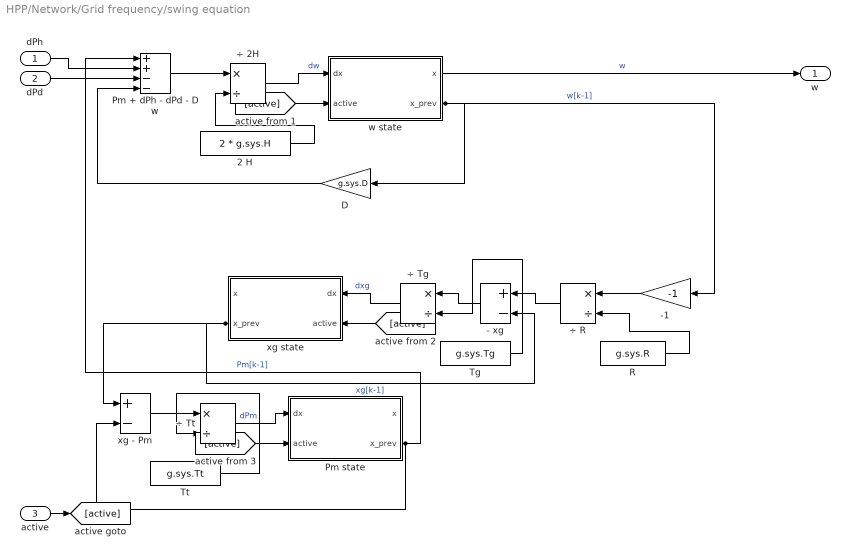
== system HPP/Network/Grid frequency/swing equation ==
  dPh : Inport
  dPd : Inport  Port=2
  active : Inport  Port=3
  - xg : Sum  Inputs=+-
  -1 : Gain  Gain=-1
  2 H : Constant  Value=2 * g.sys.H
  D : Gain  Gain=g.sys.D
  Pm + dPh - dPd - D w : Sum  Inputs=++--
  Pm state : Subsystem  Description=turbine output, forward Euler
  R : Constant  Value=g.sys.R
  Tg : Constant  Value=g.sys.Tg
  Tt : Constant  Value=g.sys.Tt
  w state : Subsystem  Description=w = w[k-1] + Ts dw while active
  xg - Pm : Sum  Inputs=+-
  xg state : Subsystem  Description=governor state, forward Euler
  ÷ 2H : Product  Inputs=*/
  ÷ R : Product  Inputs=*/
  ÷ Tg : Product  Inputs=*/
  ÷ Tt : Product  Inputs=*/
  w : Outport
  wires:
  Pm state/2(x_prev) -> Pm + dPh - dPd - D w/1, xg - Pm/2  "Pm[k-1]"
  dPh/1 -> Pm + dPh - dPd - D w/2
  dPd/1 -> Pm + dPh - dPd - D w/3
  D/1 -> Pm + dPh - dPd - D w/4
  Pm + dPh - dPd - D w/1 -> ÷ 2H/1
  2 H/1 -> ÷ 2H/2
  ÷ 2H/1 -> w state/1(dx)  "dw"
  w state/1(x) -> w/1  "w"
  w state/2(x_prev) -> D/1, -1/1  "w[k-1]"
  -1/1 -> ÷ R/1
  R/1 -> ÷ R/2
  ÷ R/1 -> - xg/1
  xg state/2(x_prev) -> - xg/2, xg - Pm/1  "xg[k-1]"
  - xg/1 -> ÷ Tg/1
  Tg/1 -> ÷ Tg/2
  ÷ Tg/1 -> xg state/1(dx)  "dxg"
  xg - Pm/1 -> ÷ Tt/1
  Tt/1 -> ÷ Tt/2
  ÷ Tt/1 -> Pm state/1(dx)  "dPm"
  active/1 -> [active]
  [active] -> w state/2(active)
  [active] -> xg state/2(active)
  [active] -> Pm state/2(active)

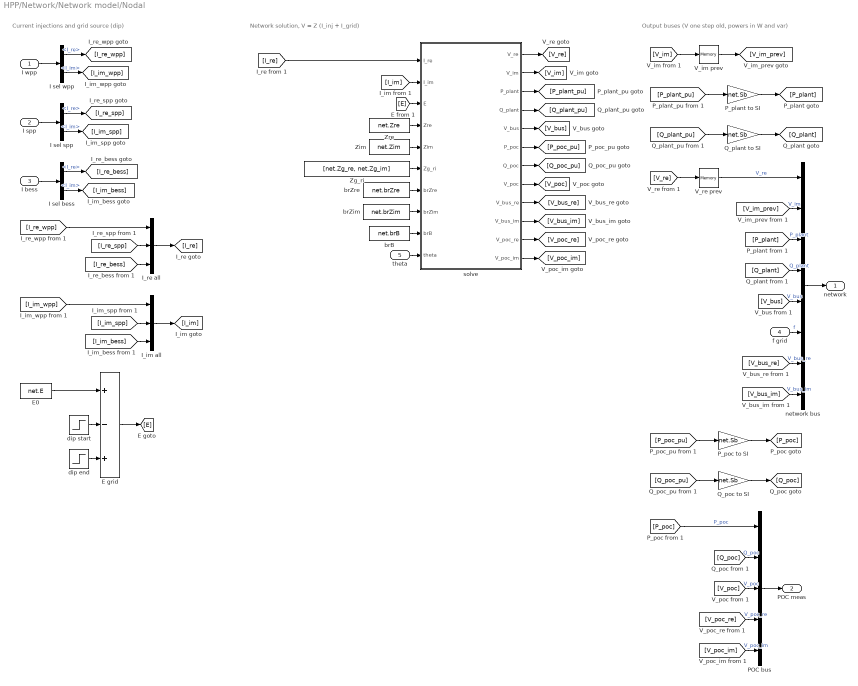
== system HPP/Network/Network model/Nodal ==
  note: Current injections and grid source (dip)
  note: Network solution, V = Z (I_inj + I_grid)
  note: Output buses (V one step old, powers in W and var)
  I wpp : Inport
  I spp : Inport  Port=2
  I bess : Inport  Port=3
  f grid : Inport  Port=4
  theta : Inport  Port=5
  E grid : Sum  Inputs=+-+
  E0 : Constant  Value=net.E
  I sel bess : BusSelector  OutputSignals=I_re,I_im
  I sel spp : BusSelector  OutputSignals=I_re,I_im
  I sel wpp : BusSelector  OutputSignals=I_re,I_im
  I_im all : Mux  Inputs=3
  I_re all : Mux  Inputs=3
  POC bus : BusCreator  Inputs=5
  P_plant to SI : Gain  Gain=net.Sb
  P_poc to SI : Gain  Gain=net.Sb
  Q_plant to SI : Gain  Gain=net.Sb
  Q_poc to SI : Gain  Gain=net.Sb
  V_im prev : Memory  InitialCondition=zeros(net.nA,1)
  V_re prev : Memory  InitialCondition=ones(net.nA,1)
  Zg_ri : Constant  Value=[net.Zg_re, net.Zg_im]
  Zim : Constant  Value=net.Zim
  Zre : Constant  Value=net.Zre
  brB : Constant  Value=net.brB
  brZim : Constant  Value=net.brZim
  brZre : Constant  Value=net.brZre
  dip end : Step  Time=p.grid.dip.t0 + p.grid.dip.dur  FinalValue=p.grid.dip.depth  SampleTime=0
  dip start : Step  Time=p.grid.dip.t0  FinalValue=p.grid.dip.depth  SampleTime=0
  network bus : BusCreator  Inputs=8
  solve : MATLAB Function  TreatAsAtomicUnit=on
  network : Outport
  POC meas : Outport  Port=2
  wires:
  I wpp/1 -> I sel wpp/1
  I sel wpp/2 -> [I_im_wpp]  "<I_im>"
  I sel wpp/1 -> [I_re_wpp]  "<I_re>"
  I spp/1 -> I sel spp/1
  I sel spp/2 -> [I_im_spp]  "<I_im>"
  I sel spp/1 -> [I_re_spp]  "<I_re>"
  I bess/1 -> I sel bess/1
  I sel bess/2 -> [I_im_bess]  "<I_im>"
  I sel bess/1 -> [I_re_bess]  "<I_re>"
  [I_re_wpp] -> I_re all/1
  [I_re_spp] -> I_re all/2
  [I_re_bess] -> I_re all/3
  I_re all/1 -> [I_re]
  [I_im_wpp] -> I_im all/1
  [I_im_spp] -> I_im all/2
  [I_im_bess] -> I_im all/3
  I_im all/1 -> [I_im]
  E0/1 -> E grid/1
  dip start/1 -> E grid/2
  dip end/1 -> E grid/3
  E grid/1 -> [E]
  [I_re] -> solve/1(I_re)
  [I_im] -> solve/2(I_im)
  [E] -> solve/3(E)
  Zre/1 -> solve/4(Zre)
  Zim/1 -> solve/5(Zim)
  Zg_ri/1 -> solve/6(Zg_ri)
  brZre/1 -> solve/7(brZre)
  brZim/1 -> solve/8(brZim)
  brB/1 -> solve/9(brB)
  theta/1 -> solve/10(theta)
  solve/2(V_im) -> [V_im]
  solve/3(P_plant) -> [P_plant_pu]
  solve/4(Q_plant) -> [Q_plant_pu]
  solve/5(V_bus) -> [V_bus]
  solve/6(P_poc) -> [P_poc_pu]
  solve/7(Q_poc) -> [Q_poc_pu]
  solve/8(V_poc) -> [V_poc]
  solve/9(V_bus_re) -> [V_bus_re]
  solve/10(V_bus_im) -> [V_bus_im]
  solve/11(V_poc_re) -> [V_poc_re]
  solve/12(V_poc_im) -> [V_poc_im]
  solve/1(V_re) -> [V_re]
  [V_im] -> V_im prev/1
  V_im prev/1 -> [V_im_prev]
  [P_plant_pu] -> P_plant to SI/1
  P_plant to SI/1 -> [P_plant]
  [Q_plant_pu] -> Q_plant to SI/1
  Q_plant to SI/1 -> [Q_plant]
  [V_re] -> V_re prev/1
  V_re prev/1 -> network bus/1  "V_re"
  [V_im_prev] -> network bus/2  "V_im"
  [P_plant] -> network bus/3  "P_plant"
  [Q_plant] -> network bus/4  "Q_plant"
  [V_bus] -> network bus/5  "V_bus"
  f grid/1 -> network bus/6  "f"
  [V_bus_re] -> network bus/7  "V_bus_re"
  [V_bus_im] -> network bus/8  "V_bus_im"
  network bus/1 -> network/1
  [P_poc_pu] -> P_poc to SI/1
  P_poc to SI/1 -> [P_poc]
  [Q_poc_pu] -> Q_poc to SI/1
  Q_poc to SI/1 -> [Q_poc]
  [P_poc] -> POC bus/1  "P_poc"
  [Q_poc] -> POC bus/2  "Q_poc"
  [V_poc] -> POC bus/3  "V_poc"
  [V_poc_re] -> POC bus/4  "V_poc_re"
  [V_poc_im] -> POC bus/5  "V_poc_im"
  POC bus/1 -> POC meas/1
